simulink model "foc_im_blocks"  (R2024b)
settings: Solver=ode23tb  StartTime=0.0  StopTime=P.T_end  MaxStep=1e-4  RelTol=1e-4
undefined symbols (not defined in the file or in its folder): P
settings Model: Creator=khali  LastModifiedBy=Khalil

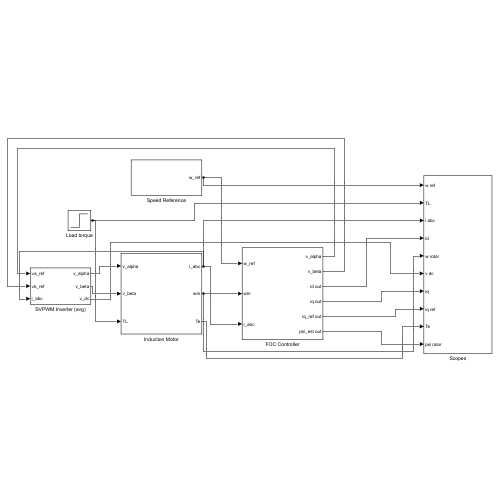
[thumbnail: Simulink's stored preview of the top-level diagram]
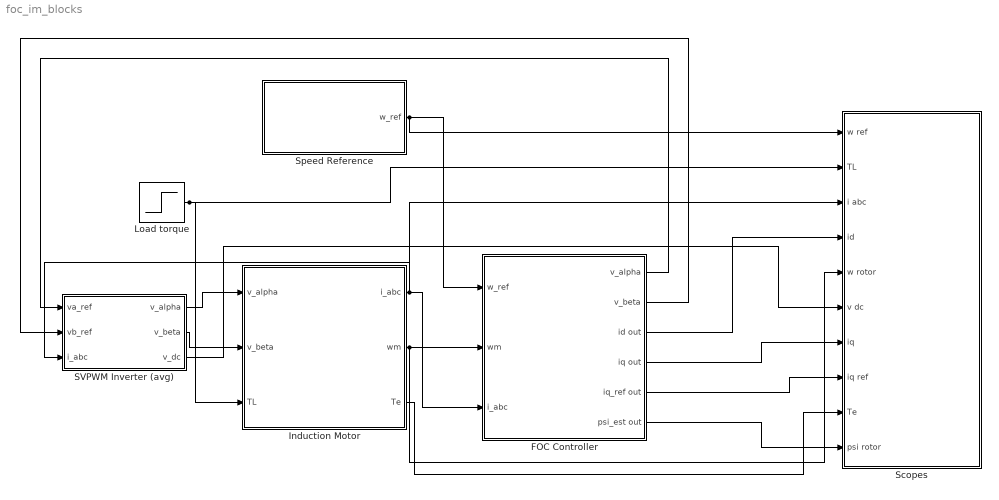
== system foc_im_blocks ==
  FOC Controller : Subsystem
  Induction Motor : Subsystem
  Load torque : Step  Time=P.t_load  After=P.TL  SampleTime=0
  SVPWM Inverter (avg) : Subsystem
  Scopes : Subsystem
  Speed Reference : Subsystem
  wires:
  FOC Controller/1(v_alpha) -> SVPWM Inverter (avg)/1(va_ref)
  SVPWM Inverter (avg)/2(v_beta) -> Induction Motor/2(v_beta)
  Load torque/1 -> Induction Motor/3(TL), Scopes/2(TL)
  SVPWM Inverter (avg)/1(v_alpha) -> Induction Motor/1(v_alpha)
  Speed Reference/1(w_ref) -> FOC Controller/1(w_ref), Scopes/1(w ref)
  Induction Motor/1(i_abc) -> SVPWM Inverter (avg)/3(i_abc), FOC Controller/3(i_abc), Scopes/3(i abc)
  Induction Motor/2(wm) -> FOC Controller/2(wm), Scopes/5(w rotor)
  FOC Controller/2(v_beta) -> SVPWM Inverter (avg)/2(vb_ref)
  FOC Controller/3(id out) -> Scopes/4(id)
  SVPWM Inverter (avg)/3(v_dc) -> Scopes/6(v dc)
  FOC Controller/4(iq out) -> Scopes/7(iq)
  FOC Controller/5(iq_ref out) -> Scopes/8(iq ref)
  Induction Motor/3(Te) -> Scopes/9(Te)
  FOC Controller/6(psi_est out) -> Scopes/10(psi rotor)

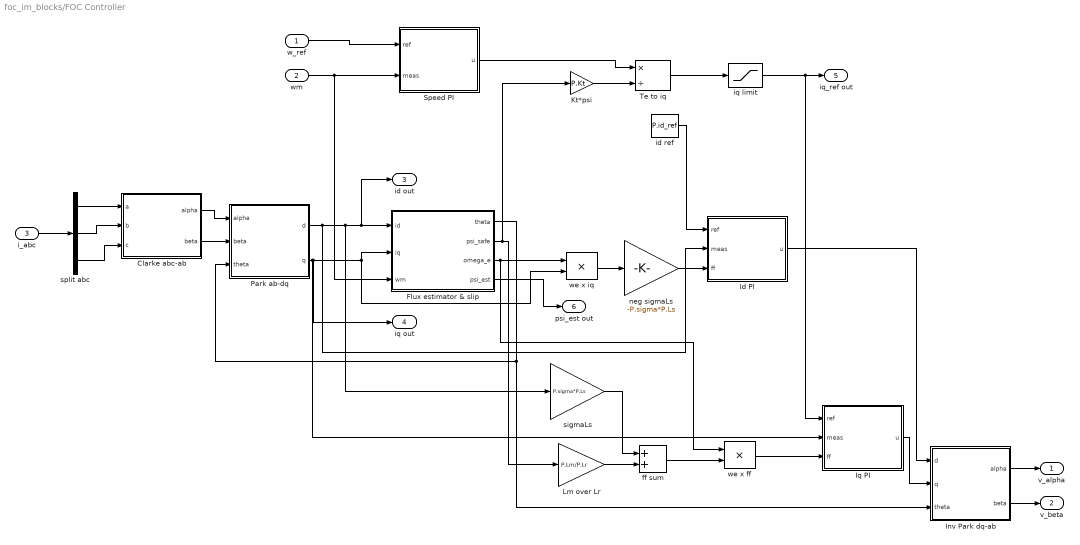
== system foc_im_blocks/FOC Controller ==
  w_ref : Inport
  wm : Inport  Port=2
  i_abc : Inport  Port=3
  Clarke abc-ab : Subsystem
  Flux estimator & slip : Subsystem
  Id PI : Subsystem
  Inv Park dq-ab : Subsystem
  Iq PI : Subsystem
  Kt*psi : Gain  Gain=P.Kt
  Lm over Lr : Gain  Gain=P.Lm/P.Lr
  Park ab-dq : Subsystem
  Speed PI : Subsystem
  Te to iq : Product  Inputs=*/
  ff sum : Sum
  id ref : Constant  Value=P.id_ref
  iq limit : Saturate  UpperLimit=P.iq_max  LowerLimit=-P.iq_max
  neg sigmaLs : Gain  Gain=-P.sigma*P.Ls
  sigmaLs : Gain  Gain=P.sigma*P.Ls
  split abc : Demux  Outputs=3
  we x ff : Product
  we x iq : Product
  v_alpha : Outport
  v_beta : Outport  Port=2
  id out : Outport  Port=3
  iq out : Outport  Port=4
  iq_ref out : Outport  Port=5
  psi_est out : Outport  Port=6
  wires:
  wm/1 -> Flux estimator & slip/3(wm), Speed PI/2(meas)
  w_ref/1 -> Speed PI/1(ref)
  i_abc/1 -> split abc/1
  split abc/3 -> Clarke abc-ab/3(c)
  Id PI/1(u) -> Inv Park dq-ab/1(d)
  split abc/2 -> Clarke abc-ab/2(b)
  split abc/1 -> Clarke abc-ab/1(a)
  Clarke abc-ab/2(beta) -> Park ab-dq/2(beta)
  Clarke abc-ab/1(alpha) -> Park ab-dq/1(alpha)
  sigmaLs/1 -> ff sum/1
  Park ab-dq/1(d) -> Flux estimator & slip/1(id), id out/1, sigmaLs/1, Id PI/2(meas)
  we x iq/1 -> neg sigmaLs/1
  Park ab-dq/2(q) -> we x iq/2, Flux estimator & slip/2(iq), iq out/1, Iq PI/2(meas)
  Speed PI/1(u) -> Te to iq/1
  Flux estimator & slip/1(theta) -> Park ab-dq/3(theta), Inv Park dq-ab/3(theta)
  Flux estimator & slip/2(psi_safe) -> Kt*psi/1, Lm over Lr/1
  Flux estimator & slip/3(omega_e) -> we x ff/1, we x iq/1
  Flux estimator & slip/4(psi_est) -> psi_est out/1
  neg sigmaLs/1 -> Id PI/3(ff)
  Kt*psi/1 -> Te to iq/2
  we x ff/1 -> Iq PI/3(ff)
  Lm over Lr/1 -> ff sum/2
  Te to iq/1 -> iq limit/1
  id ref/1 -> Id PI/1(ref)
  ff sum/1 -> we x ff/2
  iq limit/1 -> Iq PI/1(ref), iq_ref out/1
  Iq PI/1(u) -> Inv Park dq-ab/2(q)
  Inv Park dq-ab/1(alpha) -> v_alpha/1
  Inv Park dq-ab/2(beta) -> v_beta/1

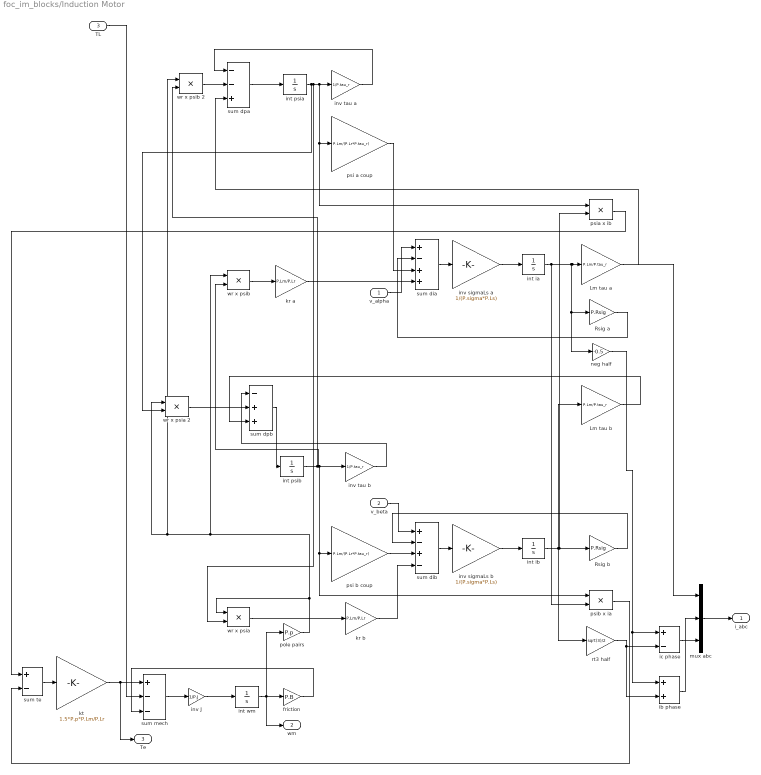
== system foc_im_blocks/Induction Motor ==
  v_alpha : Inport
  v_beta : Inport  Port=2
  TL : Inport  Port=3
  Lm tau a : Gain  Gain=P.Lm/P.tau_r
  Lm tau b : Gain  Gain=P.Lm/P.tau_r
  Rsig a : Gain  Gain=P.Rsig
  Rsig b : Gain  Gain=P.Rsig
  friction : Gain  Gain=P.B
  ib phase : Sum
  ic phase : Sum  Inputs=+-
  int ia : Integrator
  int ib : Integrator
  int psia : Integrator
  int psib : Integrator
  int wm : Integrator
  inv J : Gain  Gain=1/P.J
  inv sigmaLs a : Gain  Gain=1/(P.sigma*P.Ls)
  inv sigmaLs b : Gain  Gain=1/(P.sigma*P.Ls)
  inv tau a : Gain  Gain=1/P.tau_r
  inv tau b : Gain  Gain=1/P.tau_r
  kr a : Gain  Gain=P.Lm/P.Lr
  kr b : Gain  Gain=P.Lm/P.Lr
  kt : Gain  Gain=1.5*P.p*P.Lm/P.Lr
  mux abc : Mux  Inputs=3
  neg half : Gain  Gain=-0.5
  pole pairs : Gain  Gain=P.p
  psi a coup : Gain  Gain=P.Lm/(P.Lr*P.tau_r)
  psi b coup : Gain  Gain=P.Lm/(P.Lr*P.tau_r)
  psia x ib : Product
  psib x ia : Product
  rt3 half : Gain  Gain=sqrt(3)/2
  sum dia : Sum  Inputs=+-++
  sum dib : Sum  Inputs=+-+-
  sum dpa : Sum  Inputs=--+
  sum dpb : Sum  Inputs=-++
  sum mech : Sum  Inputs=+--
  sum te : Sum  Inputs=+-
  wr x psia : Product
  wr x psia 2 : Product
  wr x psib : Product
  wr x psib 2 : Product
  i_abc : Outport
  wm : Outport  Port=2
  Te : Outport  Port=3
  wires:
  inv J/1 -> int wm/1
  sum dpa/1 -> int psia/1
  Lm tau a/1 -> sum dpa/3
  sum mech/1 -> inv J/1
  sum dpb/1 -> int psib/1
  sum te/1 -> kt/1
  inv sigmaLs b/1 -> int ib/1
  psi b coup/1 -> sum dib/3
  TL/1 -> sum mech/2
  wr x psia 2/1 -> sum dpb/2
  wr x psib 2/1 -> sum dpa/2
  kt/1 -> sum mech/1, Te/1
  sum dib/1 -> inv sigmaLs b/1
  wr x psib/1 -> kr a/1
  Rsig a/1 -> sum dia/2
  wr x psia/1 -> kr b/1
  int wm/1 -> friction/1, wm/1, pole pairs/1
  int psia/1 -> psia x ib/1, psi a coup/1, inv tau a/1, wr x psia/2, wr x psia 2/2
  kr a/1 -> sum dia/4
  pole pairs/1 -> wr x psia 2/1, wr x psib 2/1, wr x psib/1, wr x psia/1
  int psib/1 -> psi b coup/1, psib x ia/1, inv tau b/1, wr x psib/2, wr x psib 2/2
  friction/1 -> sum mech/3
  inv tau a/1 -> sum dpa/1
  inv sigmaLs a/1 -> int ia/1
  kr b/1 -> sum dib/4
  psi a coup/1 -> sum dia/3
  int ia/1 -> mux abc/1, Lm tau a/1, neg half/1, Rsig a/1, psib x ia/2
  v_alpha/1 -> sum dia/1
  inv tau b/1 -> sum dpb/1
  Rsig b/1 -> sum dib/2
  v_beta/1 -> sum dib/1
  sum dia/1 -> inv sigmaLs a/1
  int ib/1 -> Rsig b/1, psia x ib/2, Lm tau b/1, rt3 half/1
  psia x ib/1 -> sum te/1
  neg half/1 -> ib phase/1, ic phase/1
  psib x ia/1 -> sum te/2
  Lm tau b/1 -> sum dpb/3
  mux abc/1 -> i_abc/1
  rt3 half/1 -> ib phase/2, ic phase/2
  ic phase/1 -> mux abc/3
  ib phase/1 -> mux abc/2

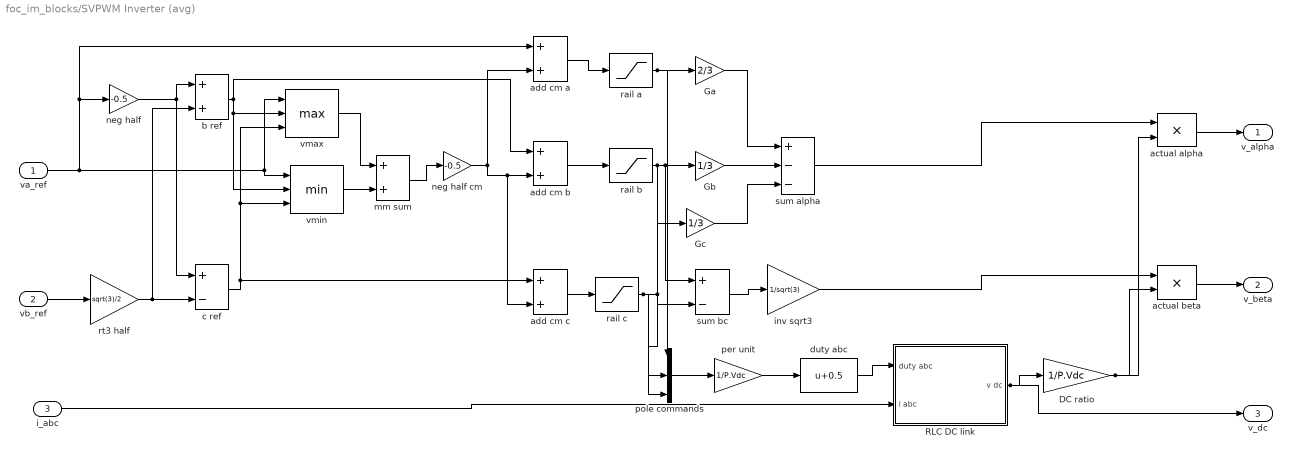
== system foc_im_blocks/SVPWM Inverter (avg) ==
  va_ref : Inport
  vb_ref : Inport  Port=2
  i_abc : Inport  Port=3
  DC ratio : Gain  Gain=1/P.Vdc
  Ga : Gain  Gain=2/3
  Gb : Gain  Gain=1/3
  Gc : Gain  Gain=1/3
  RLC DC link : Subsystem
  actual alpha : Product
  actual beta : Product
  add cm a : Sum
  add cm b : Sum
  add cm c : Sum
  b ref : Sum
  c ref : Sum  Inputs=+-
  duty abc : Bias  Bias=0.5  SaturateOnIntegerOverflow=off
  inv sqrt3 : Gain  Gain=1/sqrt(3)
  mm sum : Sum
  neg half : Gain  Gain=-0.5
  neg half cm : Gain  Gain=-0.5
  per unit : Gain  Gain=1/P.Vdc
  pole commands : Mux  Inputs=3
  rail a : Saturate  UpperLimit=P.Vdc/2  LowerLimit=-P.Vdc/2
  rail b : Saturate  UpperLimit=P.Vdc/2  LowerLimit=-P.Vdc/2
  rail c : Saturate  UpperLimit=P.Vdc/2  LowerLimit=-P.Vdc/2
  rt3 half : Gain  Gain=sqrt(3)/2
  sum alpha : Sum  Inputs=+--
  sum bc : Sum  Inputs=+-
  vmax : MinMax  Function=max  Inputs=3
  vmin : MinMax  Inputs=3
  v_alpha : Outport
  v_beta : Outport  Port=2
  v_dc : Outport  Port=3
  wires:
  rt3 half/1 -> b ref/2, c ref/2
  c ref/1 -> add cm c/1, vmax/3, vmin/3
  vmin/1 -> mm sum/2
  vmax/1 -> mm sum/1
  b ref/1 -> vmin/2, vmax/2, add cm b/1
  neg half/1 -> b ref/1, c ref/1
  vb_ref/1 -> rt3 half/1
  va_ref/1 -> vmax/1, vmin/1, add cm a/1, neg half/1
  rail c/1 -> sum bc/2, Gc/1, pole commands/3
  mm sum/1 -> neg half cm/1
  Ga/1 -> sum alpha/1
  neg half cm/1 -> add cm b/2, add cm c/2, add cm a/2
  add cm a/1 -> rail a/1
  add cm b/1 -> rail b/1
  add cm c/1 -> rail c/1
  rail a/1 -> Ga/1, pole commands/1
  rail b/1 -> Gb/1, sum bc/1, pole commands/2
  Gb/1 -> sum alpha/2
  Gc/1 -> sum alpha/3
  sum bc/1 -> inv sqrt3/1
  pole commands/1 -> per unit/1
  per unit/1 -> duty abc/1
  duty abc/1 -> RLC DC link/1(duty abc)
  i_abc/1 -> RLC DC link/2(i abc)
  RLC DC link/1(v dc) -> DC ratio/1, v_dc/1
  sum alpha/1 -> actual alpha/1
  inv sqrt3/1 -> actual beta/1
  DC ratio/1 -> actual alpha/2, actual beta/2
  actual alpha/1 -> v_alpha/1
  actual beta/1 -> v_beta/1

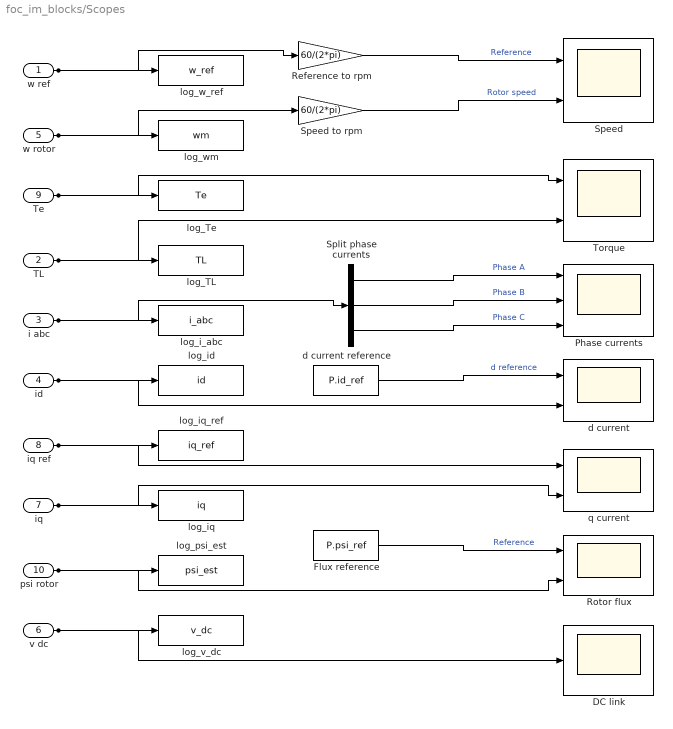
== system foc_im_blocks/Scopes ==
  w ref : Inport
  TL : Inport  Port=2
  i abc : Inport  Port=3
  id : Inport  Port=4
  w rotor : Inport  Port=5
  v dc : Inport  Port=6
  iq : Inport  Port=7
  iq ref : Inport  Port=8
  Te : Inport  Port=9
  psi rotor : Inport  Port=10
  DC link : Scope
  Flux reference : Constant  Value=P.psi_ref
  Phase currents : Scope  NumInputPorts=3
  Reference to rpm : Gain  Gain=60/(2*pi)
  Rotor flux : Scope  NumInputPorts=2
  Speed : Scope  NumInputPorts=2
  Speed to rpm : Gain  Gain=60/(2*pi)
  Split phase currents : Demux  Outputs=3
  Torque : Scope  NumInputPorts=2
  d current : Scope  NumInputPorts=2
  d current reference : Constant  Value=P.id_ref
  log_TL : ToWorkspace  VariableName=TL  SaveFormat=Timeseries  SampleTime=-1
  log_Te : ToWorkspace  VariableName=Te  SaveFormat=Timeseries  SampleTime=-1
  log_i_abc : ToWorkspace  VariableName=i_abc  SaveFormat=Timeseries  SampleTime=-1
  log_id : ToWorkspace  VariableName=id  SaveFormat=Timeseries  SampleTime=-1
  log_iq : ToWorkspace  VariableName=iq  SaveFormat=Timeseries  SampleTime=-1
  log_iq_ref : ToWorkspace  VariableName=iq_ref  SaveFormat=Timeseries  SampleTime=-1
  log_psi_est : ToWorkspace  VariableName=psi_est  SaveFormat=Timeseries  SampleTime=-1
  log_v_dc : ToWorkspace  VariableName=v_dc  SaveFormat=Timeseries  SampleTime=-1
  log_w_ref : ToWorkspace  VariableName=w_ref  SaveFormat=Timeseries  SampleTime=-1
  log_wm : ToWorkspace  VariableName=wm  SaveFormat=Timeseries  SampleTime=-1
  q current : Scope  NumInputPorts=2
  wires:
  w ref/1 -> log_w_ref/1, Reference to rpm/1
  TL/1 -> log_TL/1, Torque/2
  i abc/1 -> log_i_abc/1, Split phase currents/1
  id/1 -> log_id/1, d current/2
  w rotor/1 -> log_wm/1, Speed to rpm/1
  v dc/1 -> log_v_dc/1, DC link/1
  iq/1 -> log_iq/1, q current/2
  iq ref/1 -> log_iq_ref/1, q current/1
  Te/1 -> log_Te/1, Torque/1
  psi rotor/1 -> log_psi_est/1, Rotor flux/2
  Reference to rpm/1 -> Speed/1  "Reference"
  Speed to rpm/1 -> Speed/2  "Rotor speed"
  Split phase currents/1 -> Phase currents/1  "Phase A"
  Split phase currents/2 -> Phase currents/2  "Phase B"
  Split phase currents/3 -> Phase currents/3  "Phase C"
  d current reference/1 -> d current/1  "d reference"
  Flux reference/1 -> Rotor flux/1  "Reference"

== system foc_im_blocks/Speed Reference ==
  staircase : Sum  Inputs=++++
  step1 : Step  Time=P.step_t(1)  After=P.step_d(1)  SampleTime=0
  step2 : Step  Time=P.step_t(2)  After=P.step_d(2)  SampleTime=0
  step3 : Step  Time=P.step_t(3)  After=P.step_d(3)  SampleTime=0
  step4 : Step  Time=P.step_t(4)  After=P.step_d(4)  SampleTime=0
  w_ref : Outport
  wires:
  step3/1 -> staircase/3
  step2/1 -> staircase/2
  step1/1 -> staircase/1
  staircase/1 -> w_ref/1
  step4/1 -> staircase/4

== system foc_im_blocks/FOC Controller/Clarke abc-ab ==
  a : Inport
  b : Inport  Port=2
  c : Inport  Port=3
  Ga : Gain  Gain=2/3
  Gb : Gain  Gain=1/3
  Gc : Gain  Gain=1/3
  inv sqrt3 : Gain  Gain=1/sqrt(3)
  sum alpha : Sum  Inputs=+--
  sum bc : Sum  Inputs=+-
  alpha : Outport
  beta : Outport  Port=2
  wires:
  c/1 -> Gc/1, sum bc/2
  b/1 -> Gb/1, sum bc/1
  a/1 -> Ga/1
  Gc/1 -> sum alpha/3
  sum alpha/1 -> alpha/1
  Gb/1 -> sum alpha/2
  Ga/1 -> sum alpha/1
  sum bc/1 -> inv sqrt3/1
  inv sqrt3/1 -> beta/1

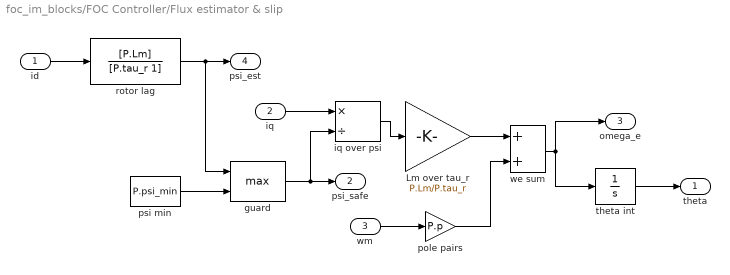
== system foc_im_blocks/FOC Controller/Flux estimator & slip ==
  id : Inport
  iq : Inport  Port=2
  wm : Inport  Port=3
  Lm over tau_r : Gain  Gain=P.Lm/P.tau_r
  guard : MinMax  Function=max  Inputs=2
  iq over psi : Product  Inputs=*/
  pole pairs : Gain  Gain=P.p
  psi min : Constant  Value=P.psi_min
  rotor lag : TransferFcn  Numerator=[P.Lm]  Denominator=[P.tau_r 1]
  theta int : Integrator
  we sum : Sum
  theta : Outport
  psi_safe : Outport  Port=2
  omega_e : Outport  Port=3
  psi_est : Outport  Port=4
  wires:
  wm/1 -> pole pairs/1
  iq/1 -> iq over psi/1
  id/1 -> rotor lag/1
  psi min/1 -> guard/2
  rotor lag/1 -> guard/1, psi_est/1
  Lm over tau_r/1 -> we sum/1
  theta int/1 -> theta/1
  iq over psi/1 -> Lm over tau_r/1
  guard/1 -> iq over psi/2, psi_safe/1
  pole pairs/1 -> we sum/2
  we sum/1 -> omega_e/1, theta int/1

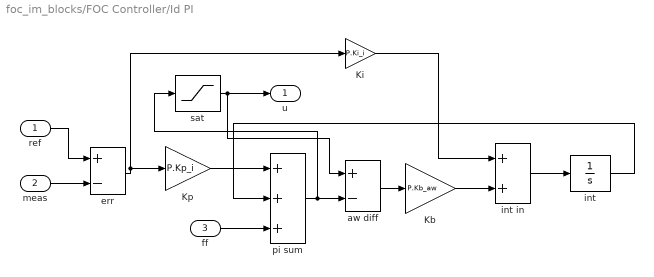
== system foc_im_blocks/FOC Controller/Id PI ==
  ref : Inport
  meas : Inport  Port=2
  ff : Inport  Port=3
  Kb : Gain  Gain=P.Kb_aw
  Ki : Gain  Gain=P.Ki_i
  Kp : Gain  Gain=P.Kp_i
  aw diff : Sum  Inputs=+-
  err : Sum  Inputs=+-
  int : Integrator  LimitOutput=on  UpperSaturationLimit=P.v_max  LowerSaturationLimit=-P.v_max
  int in : Sum
  pi sum : Sum  Inputs=+++
  sat : Saturate  UpperLimit=P.v_max  LowerLimit=-P.v_max
  u : Outport
  wires:
  Ki/1 -> int in/1
  pi sum/1 -> sat/1, aw diff/2
  ff/1 -> pi sum/3
  meas/1 -> err/2
  Kp/1 -> pi sum/1
  ref/1 -> err/1
  err/1 -> Ki/1, Kp/1
  sat/1 -> aw diff/1, u/1
  aw diff/1 -> Kb/1
  Kb/1 -> int in/2
  int in/1 -> int/1
  int/1 -> pi sum/2

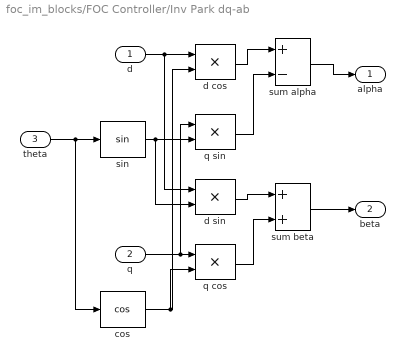
== system foc_im_blocks/FOC Controller/Inv Park dq-ab ==
  d : Inport
  q : Inport  Port=2
  theta : Inport  Port=3
  cos : Trigonometry  Operator=cos
  d cos : Product
  d sin : Product
  q cos : Product
  q sin : Product
  sin : Trigonometry
  sum alpha : Sum  Inputs=+-
  sum beta : Sum
  alpha : Outport
  beta : Outport  Port=2
  wires:
  d cos/1 -> sum alpha/1
  d sin/1 -> sum beta/1
  q cos/1 -> sum beta/2
  sin/1 -> q sin/2, d sin/2
  q sin/1 -> sum alpha/2
  cos/1 -> d cos/2, q cos/2
  q/1 -> q sin/1, q cos/1
  theta/1 -> cos/1, sin/1
  d/1 -> d cos/1, d sin/1
  sum alpha/1 -> alpha/1
  sum beta/1 -> beta/1

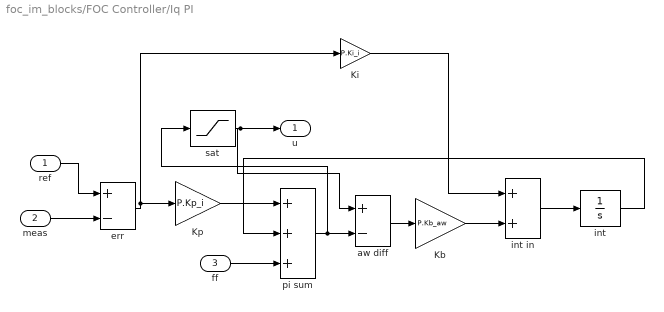
== system foc_im_blocks/FOC Controller/Iq PI ==
  ref : Inport
  meas : Inport  Port=2
  ff : Inport  Port=3
  Kb : Gain  Gain=P.Kb_aw
  Ki : Gain  Gain=P.Ki_i
  Kp : Gain  Gain=P.Kp_i
  aw diff : Sum  Inputs=+-
  err : Sum  Inputs=+-
  int : Integrator  LimitOutput=on  UpperSaturationLimit=P.v_max  LowerSaturationLimit=-P.v_max
  int in : Sum
  pi sum : Sum  Inputs=+++
  sat : Saturate  UpperLimit=P.v_max  LowerLimit=-P.v_max
  u : Outport
  wires:
  Ki/1 -> int in/1
  pi sum/1 -> sat/1, aw diff/2
  ff/1 -> pi sum/3
  meas/1 -> err/2
  Kp/1 -> pi sum/1
  ref/1 -> err/1
  err/1 -> Ki/1, Kp/1
  sat/1 -> aw diff/1, u/1
  aw diff/1 -> Kb/1
  Kb/1 -> int in/2
  int in/1 -> int/1
  int/1 -> pi sum/2

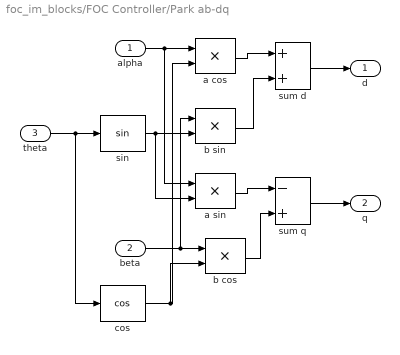
== system foc_im_blocks/FOC Controller/Park ab-dq ==
  alpha : Inport
  beta : Inport  Port=2
  theta : Inport  Port=3
  a cos : Product
  a sin : Product
  b cos : Product
  b sin : Product
  cos : Trigonometry  Operator=cos
  sin : Trigonometry
  sum d : Sum
  sum q : Sum  Inputs=-+
  d : Outport
  q : Outport  Port=2
  wires:
  cos/1 -> a cos/2, b cos/2
  sin/1 -> b sin/2, a sin/2
  theta/1 -> cos/1, sin/1
  beta/1 -> b sin/1, b cos/1
  alpha/1 -> a sin/1, a cos/1
  b cos/1 -> sum q/2
  a cos/1 -> sum d/1
  b sin/1 -> sum d/2
  a sin/1 -> sum q/1
  sum q/1 -> q/1
  sum d/1 -> d/1

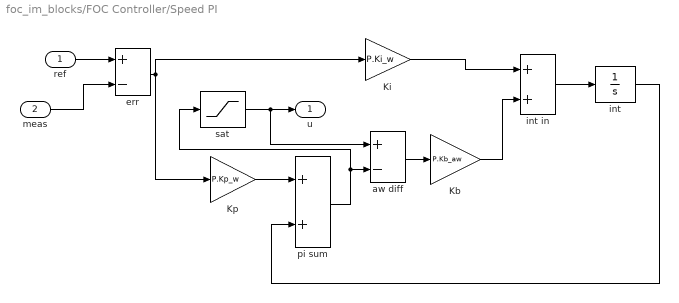
== system foc_im_blocks/FOC Controller/Speed PI ==
  ref : Inport
  meas : Inport  Port=2
  Kb : Gain  Gain=P.Kb_aw
  Ki : Gain  Gain=P.Ki_w
  Kp : Gain  Gain=P.Kp_w
  aw diff : Sum  Inputs=+-
  err : Sum  Inputs=+-
  int : Integrator  LimitOutput=on  UpperSaturationLimit=P.Te_max  LowerSaturationLimit=-P.Te_max
  int in : Sum
  pi sum : Sum
  sat : Saturate  UpperLimit=P.Te_max  LowerLimit=-P.Te_max
  u : Outport
  wires:
  ref/1 -> err/1
  Ki/1 -> int in/1
  pi sum/1 -> sat/1, aw diff/2
  meas/1 -> err/2
  Kp/1 -> pi sum/1
  err/1 -> Ki/1, Kp/1
  aw diff/1 -> Kb/1
  sat/1 -> aw diff/1, u/1
  Kb/1 -> int in/2
  int in/1 -> int/1
  int/1 -> pi sum/2

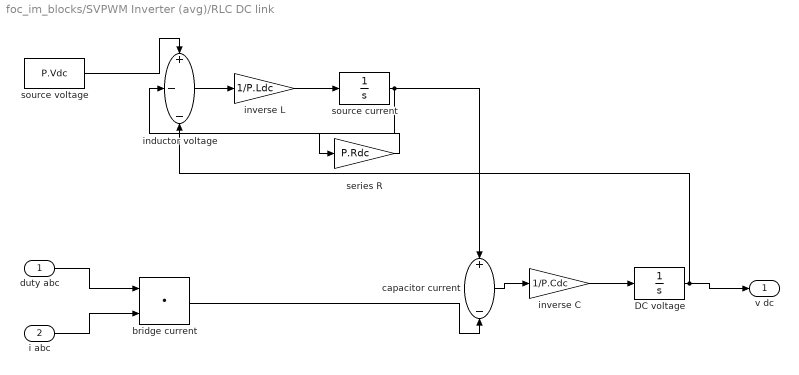
== system foc_im_blocks/SVPWM Inverter (avg)/RLC DC link ==
  duty abc : Inport
  i abc : Inport  Port=2
  DC voltage : Integrator  InitialCondition=P.Vdc
  bridge current : DotProduct  OutDataTypeStr=Inherit: Inherit via internal rule
  capacitor current : Sum  Inputs=+-
  inductor voltage : Sum  Inputs=+--
  inverse C : Gain  Gain=1/P.Cdc
  inverse L : Gain  Gain=1/P.Ldc
  series R : Gain  Gain=P.Rdc
  source current : Integrator
  source voltage : Constant  Value=P.Vdc
  v dc : Outport
  wires:
  source voltage/1 -> inductor voltage/1
  series R/1 -> inductor voltage/2
  DC voltage/1 -> inductor voltage/3, v dc/1
  inductor voltage/1 -> inverse L/1
  inverse L/1 -> source current/1
  source current/1 -> series R/1, capacitor current/1
  duty abc/1 -> bridge current/1
  i abc/1 -> bridge current/2
  bridge current/1 -> capacitor current/2
  capacitor current/1 -> inverse C/1
  inverse C/1 -> DC voltage/1
